simulink model "Controller_damping_cbf_22"  (R2022b)
settings: Solver=ode4  StartTime=0.0  StopTime=Inf  FixedStep=1e-3  RelTol=1e-3
values from neighbouring files (symbols this model uses):
  cbf_damping_params = [cbf_p_ths; cbf_v_ths; cbf_v_0; cbf_gamma; cbf_d_max;                        cbf_w_lin; cbf_w_quad; plane_normal; plane_offset;                        cbf_latch_entry; cbf_zone_hyst; cbf_latch_alpha; cbf_clip_drift;                        cbf_tau_rate; cbf_dt; cbf_gamma_pos_scale]    [init_damping_cbf.m]
  Dn = 20 * ones(7,1)    [init_damping_cbf.m]
  H_0_cy = H_0_pr * H_pr_cy    [init_damping_cbf.m]
  H_home = getTransform(Franka_robot, q_home, 'panda_link8', 'panda_link0')    [init_damping_cbf.m]
  Kn = 0 * ones(7,1)    [init_damping_cbf.m]
  q_home = q_init    [init_damping_cbf.m]
  q_init = [0 0  0  -(2/4)*pi  0  pi/2  -pi/4]'    [init_damping_cbf.m]
undefined symbols (not defined in the file or in its folder): DiscIntNeverNeededParam, Fext_mag, T_final, X, Y, Z
libraries: sm_lib x162, nesl_utility x44, matrix_library x3, Robotics_lib x1
(part 7 of 12)

== matlab function Controller_damping_cbf_22/Dynamic Parameters/Mass Matrix ==
  data: q input; m output
function m = maple_R7plus_massmatrix_04(q)
% Author: TU Wien, ACIN Robotics group
% Optimized and generated from Maple
  m = zeros(7,7);
  t378 = q(6);
  t364 = sin(t378);
  t371 = cos(t378);
  t494 = 0.60149e-1 * t364 - 0.14117e-1 * t371;
  t246 = t494 + 0.384e0;
  t380 = q(4);
  t366 = sin(t380);
  t214 = t246 * t366;
  t381 = q(3);
  t374 = cos(t381);
  t269 = 0.60149e-1 * t371 + 0.14117e-1 * t364;
  t379 = q(5);
  t365 = sin(t379);
  t372 = cos(t379);
  t159 = t269 * t365 + 0.10517e-1 * t372;
  t367 = sin(t381);
  t424 = t159 * t367;
  t373 = cos(t380);
  t681 = 0.10517e-1 * t365;
  t437 = -t269 * t372 + t681;
  t906 = 0.825e-1 + t437;
  t915 = t906 * t373;
  t937 = t424 + (t214 + t915) * t374;
  t377 = q(7);
  t363 = sin(t377);
  t370 = cos(t377);
  t499 = -0.10517e-1 * t370 - 0.4252e-2 * t363;
  t254 = -t499 + 0.88e-1;
  t417 = t254 * t364 - 0.61597e-1 * t371;
  t910 = 0.384e0 + t417;
  t889 = t910 * t366;
  t472 = -0.825e-1 + t889;
  t172 = 0.10517000000000000000000000000000e-1 * t363 - 0.42520000000000000000000000000000e-2 * t370;
  t815 = t172 * t365;
  t682 = 0.61597e-1 * t364;
  t768 = t371 * t372;
  t911 = -t254 * t768 - t372 * t682 + 0.825e-1;
  t70 = -t815 + t911;
  t41 = t373 * t70 + t472;
  t802 = t254 * t371;
  t418 = t682 + t802;
  t895 = t365 * t418;
  t864 = -t172 * t372 + t895;
  t935 = t367 * t864 + t374 * t41;
  t515 = 0.12009367848960000000000000000000e-2 * t363 + 0.63347540234880000000000000000000e-1;
  t530 = 0.29704261916160000000000000000000e-2 * t370;
  t126 = t515 + t530;
  t349 = t363 ^ 2;
  t294 = 0.13297872941088000000000000000000e-4 * t349;
  t356 = t370 ^ 2;
  t328 = 0.2407645905580142000000000000000e-2 * t356;
  t305 = 0.55042935974400000000000000000000e-3 * t363;
  t514 = t305 + 0.57804776249276620000000000000000e-2;
  t459 = -t328 + t294 + t514;
  t562 = 0.79021743663150400000000000000000e-3 * t363;
  t811 = (-0.13614453378240000000000000000000e-2 + t562) * t370;
  t871 = t811 - t459;
  t59 = t871 * t364;
  t928 = -t126 + t59;
  t933 = t371 * t928;
  t916 = t906 * t366;
  t434 = 0.98827089590400000000000000000000e-3 * t363 + 0.52129746651620000000000000000000e-1;
  t138 = 0.24444132201840000000000000000000e-2 * t370 + t434;
  t832 = t138 * t364;
  t358 = t372 ^ 2;
  t316 = 0.24890000000000000000000000000000e-2 * t356;
  t799 = t363 * t370;
  t488 = 0.85600000000000000000000000000000e-3 * t799;
  t453 = t316 + t488;
  t420 = t453 - 0.27050000000000000000000000000000e-2;
  t117 = t453 + 0.28220000000000000000000000000000e-2;
  t357 = t371 ^ 2;
  t99 = t117 * t357;
  t413 = t420 + t99;
  t298 = 0.14820000000000000000000000000000e-2 * t363;
  t532 = 0.23920000000000000000000000000000e-2 * t370;
  t465 = t298 - t532;
  t163 = -t465 + 0.218e-3;
  t796 = t364 * t371;
  t734 = t163 * t796;
  t909 = t734 - t413;
  t932 = t909 * t358;
  t295 = 0.29704261916160000000000000000000e-2 * t363;
  t509 = 0.23898270415101870000000000000000e-1 - t295;
  t535 = 0.12009367848960000000000000000000e-2 * t370;
  t131 = t509 + t535;
  t318 = 0.79021743663150400000000000000000e-3 * t356;
  t238 = -0.68072266891200000000000000000000e-3 * t363 + 0.29134980109706700000000000000000e-3;
  t812 = (0.24209437785212300000000000000000e-2 * t363 + 0.27521467987200000000000000000000e-3) * t370;
  t922 = t238 + t812;
  t908 = -t318 + t922;
  t925 = t908 * t364;
  t698 = t131 + t925;
  t382 = q(2);
  t375 = cos(t382);
  t757 = t375 * t373;
  t368 = sin(t382);
  t772 = t368 * t374;
  t249 = t366 * t772 + t757;
  t804 = t249 * t371;
  t780 = t367 * t368;
  t758 = t375 * t366;
  t761 = t373 * t374;
  t242 = -0.1e1 * t368 * t761 + t758;
  t896 = t242 * t372;
  t140 = t365 * t780 + t896;
  t828 = t140 * t364;
  t919 = -0.1e1 * t828 + t804;
  t351 = t365 ^ 2;
  t792 = t365 * t372;
  t622 = 0.4234e-2 * t792;
  t931 = 0.29474e-1 * t351 + 0.35549e-1 * t358 + t622 + 0.25853e-1;
  t930 = 0.28179e-1;
  t929 = t373 - 0.1e1;
  t927 = t159 * t374;
  t781 = t366 * t374;
  t692 = 0.4252e-2 * t370;
  t500 = 0.10517e-1 * t363 - t692;
  t456 = t500 * t372;
  t399 = t456 - t895;
  t926 = t399 * t367;
  t924 = t908 * t365;
  t923 = t908 * t371;
  t344 = 0.345563e0 * t366;
  t329 = -0.825e-1 + t344;
  t493 = 0.41065e-1 * t365 + 0.11953e-1 * t372;
  t247 = t493 + 0.825e-1;
  t805 = t247 * t373;
  t142 = t329 + t805;
  t173 = -0.41065000000000000000000000000000e-1 * t372 + 0.11953000000000000000000000000000e-1 * t365;
  t73 = t142 * t367 + t173 * t374;
  t748 = t294 + t305;
  t921 = -0.32797153116247448000000000000000e-1 - t748 + t811;
  t383 = q(1);
  t376 = cos(t383);
  t756 = t375 * t376;
  t719 = t367 * t756;
  t369 = sin(t383);
  t770 = t369 * t374;
  t920 = -t719 - t770;
  t725 = t372 * t780;
  t808 = t242 * t365;
  t124 = t808 - 0.1e1 * t725;
  t807 = t246 * t373;
  t918 = t366 * t437 - t807;
  t917 = t59 - t515;
  t304 = 0.63817750210500000000000000000000e-3 * t363;
  t542 = 0.25801376238000000000000000000000e-3 * t370;
  t433 = 0.55993270925625000000000000000000e-2 + t542;
  t127 = -t304 + t433;
  t106 = t127 * t373;
  t540 = 0.54835910640823200000000000000000e-3 * t370;
  t560 = 0.16724826617837780000000000000000e-2 * t363;
  t175 = -t540 - t560;
  t141 = -t175 + 0.9356909731460500000000000000000e-4;
  t824 = t141 * t371;
  t226 = 0.56786982094425000000000000000000e-2 * t364 - 0.12089329343850000000000000000000e-2;
  t183 = t226 * t373;
  t793 = t365 * t371;
  t912 = -0.24076459055801420000000000000000e-2 * t356 - t811;
  t58 = (-0.89033153705875550000000000000000e-2 - t748 - t912) * t357;
  t299 = 0.12763550042100000000000000000000e-2 * t363;
  t541 = 0.51602752476000000000000000000000e-3 * t370;
  t432 = 0.11198654185125000000000000000000e-1 + t541;
  t882 = t299 - t432;
  t891 = t882 * t365;
  t559 = 0.23920000000000000000000000000000e-2 * t363;
  t259 = 0.682e-3 + t559;
  t533 = 0.14820000000000000000000000000000e-2 * t370;
  t265 = t364 * t533;
  t486 = 0.49780000000000000000000000000000e-2 * t799;
  t426 = 0.14600000000000000000000000000000e-2 - t486;
  t565 = 0.17120000000000000000000000000000e-2 * t356;
  t119 = t426 + t565;
  t840 = t119 * t371;
  t914 = t259 * t364 + t265 + t840;
  t700 = 0.825e-1 * t366;
  t704 = 0.825e-1 * t375;
  t913 = t368 * t700 + t704 * t761;
  t68 = t328 + t921;
  t487 = 0.24890000000000000000000000000000e-2 * t799;
  t567 = 0.85600000000000000000000000000000e-3 * t356;
  t116 = t487 - 0.73000000000000000000000000000000e-3 - t567;
  t538 = 0.74100000000000000000000000000000e-3 * t370;
  t483 = t364 * t538;
  t54 = -0.4234e-2 + t914;
  t451 = -0.11960000000000000000000000000000e-2 * t363 - 0.341e-3;
  t686 = t451 * t364 + 0.3449e-2;
  t907 = t116 * t371 + t358 * t54 - t792 * t909 - t483 + t686;
  t400 = -t365 * t500 - t372 * t418;
  t215 = 0.48418875570424600000000000000000e-2 * t363 + 0.55042935974400000000000000000000e-3;
  t561 = 0.13614453378240000000000000000000e-2 * t363;
  t566 = 0.15804348732630080000000000000000e-2 * t356;
  t87 = t215 * t370 - t561 - t566 + 0.5826996021941340000000000000000e-3;
  t78 = t87 * t371;
  t580 = -0.3030488946654060e-2 - t78;
  t534 = 0.12763550042100000000000000000000e-2 * t370;
  t310 = 0.11357396418885000000000000000000e-1 * t364;
  t513 = t310 - 0.24178658687700000000000000000000e-2;
  t313 = 0.56786982094425000000000000000000e-2 * t366;
  t422 = t313 - 0.21751134959804000000000000000000e-1 * t373;
  t306 = 0.54835910640823200000000000000000e-3 * t363;
  t511 = 0.44842466056464210000000000000000e-2 - t306;
  t548 = 0.12089329343850000000000000000000e-2 * t366;
  t904 = 0.46305794820080000000000000000000e-2 * t373 - t511 - t548 + (t422 - 0.26431758938496000000000000000000e-1) * t364;
  t350 = t364 ^ 2;
  t308 = 0.31228377456598930000000000000000e-2 * t350;
  t564 = 0.25022978729410880000000000000000e-2 * t356;
  t427 = t308 + 0.6284682367054690000000000000000e-3 - t564;
  t264 = t370 * t562;
  t293 = 0.81354094419858000000000000000000e-4 * t349;
  t751 = t264 + t293;
  t79 = -t427 + t751;
  t903 = t58 + t79;
  t901 = t54 * t792;
  t572 = 0.2489000000000000000000000000000e-2 * t356;
  t415 = -t488 - t572;
  t120 = -t415 + 0.28220000000000000000000000000000e-2;
  t327 = 0.4978000000000000000000000000000e-2 * t356;
  t263 = 0.17120000000000000000000000000000e-2 * t799;
  t508 = 0.33106000000000000000000000000000e-1 - t263;
  t46 = -t120 * t357 + t327 - t508 + t734;
  t854 = t901 + t932;
  t900 = t46 + t854;
  t169 = -0.825e-1 + t214;
  t884 = t169 + t915;
  t899 = t374 * t884 + t424;
  t537 = 0.10967182128164640000000000000000e-2 * t370;
  t558 = 0.33449653235675560000000000000000e-2 * t363;
  t423 = t537 + t558;
  t405 = t423 + 0.18713819462921000000000000000000e-3;
  t898 = -t364 * t405 - t580;
  t464 = 0.33449653235675560000000000000000e-2 * t370 - 0.10967182128164640000000000000000e-2 * t363;
  t128 = 0.11022068765350630000000000000000e-1 + t464;
  t108 = t128 * t357;
  t555 = 0.88000000000000000000000000000000e-1 * t364;
  t224 = 0.38400000000000000000000000000000e0 + t555;
  t897 = t224 * t367;
  t490 = -0.104419e0 * t373 + 0.5317e-1 * t366;
  t893 = t368 * t490;
  t645 = 0.345563e0 * t373;
  t806 = t247 * t366;
  t576 = -t645 + t806;
  t892 = t368 * t576;
  t721 = t374 * t756;
  t779 = t367 * t369;
  t503 = t373 * (t721 - 0.1e1 * t779);
  t890 = (t576 - 0.316e0) * t375;
  t822 = t910 * t373;
  t222 = -t304 + 0.55993270925625000000000000000000e-2;
  t888 = (t222 + t542) * t373;
  t492 = -0.41065e-1 * t372 + 0.11953e-1 * t365;
  t887 = t492 * t367;
  t623 = 0.7735484874e-2 * t370;
  t154 = (0.76800000000000000000000000000000e0 * t364 + 0.17600000000000000000000000000000e0) * t623;
  t231 = 0.24018735697920000000000000000000e-2 * t363 + 0.12669508046976000000000000000000e0;
  t885 = t231 * t364 + t154;
  t326 = 0.54835910640823200000000000000000e-3 * t374;
  t543 = 0.24444132201840000000000000000000e-2 * t367;
  t881 = t326 + t543;
  t595 = 0.2964e-2 * t363 - 0.4784e-2 * t370 - 0.436e-3;
  t880 = -0.1e1 * t328 - 0.26431758938496000000000000000000e-1 * t371 - t921;
  t879 = t363 * t681 - t365 * t692 - t911;
  t877 = t514 + t912;
  t648 = 0.249498e0 * t368;
  t679 = 0.39252e-1 * t367;
  t876 = -t375 * t679 + t648;
  t627 = 0.3127439544e-2 * t363;
  t875 = t623 + t627;
  t874 = 0.88e-1 * t371 + t682;
  t740 = t128 * t796;
  t873 = t740 - t58;
  t870 = t58 - 0.1e1 * t740;
  t258 = -0.74100000000000000000000000000000e-3 * t363 + 0.4146e-2;
  t536 = 0.11960000000000000000000000000000e-2 * t370;
  t737 = t120 * t796;
  t818 = t163 * t357;
  t439 = -t536 + t737 + t818;
  t869 = -0.1e1 * t258 + t439;
  t568 = t263 + 0.5644000000000000000000000000000e-2;
  t121 = t327 + t568;
  t736 = t121 * t796;
  t463 = -0.47840000000000000000000000000000e-2 * t370 + 0.29640000000000000000000000000000e-2 * t363;
  t162 = t463 - 0.436e-3;
  t819 = t162 * t357;
  t867 = t736 - 0.1e1 * t819;
  t322 = 0.13614453378240000000000000000000e-2 * t370;
  t866 = -0.1e1 * t305 - 0.1e1 * t322;
  t649 = 0.104419e0 * t366;
  t491 = 0.5317e-1 * t373 + t649;
  t248 = t491 - 0.825e-1;
  t442 = t248 * t367;
  t669 = 0.27454e-1 * t374;
  t865 = (t442 + t669) * t376;
  t863 = 0.735522e0 * t369;
  t647 = 0.735522e0 * t371;
  t657 = 0.27518e-1 * t369;
  t660 = 0.39252e-1 * t376;
  t862 = t376 * t648 + (-t375 * t660 - t657) * t367;
  t795 = t364 * t372;
  t861 = -t116 * t795 - 0.8641e-2;
  t860 = 0.1225946e1 * t73;
  t296 = 0.24444132201840000000000000000000e-2 * t363;
  t431 = 0.98827089590400000000000000000000e-3 * t370 + 0.21447119530300000000000000000000e-1;
  t139 = -t296 + t431;
  t225 = -0.21751134959804000000000000000000e-1 * t364 + 0.46305794820080000000000000000000e-2;
  t859 = t139 * t365 + (-0.1e1 * t138 * t371 + t225) * t372;
  t858 = 0.25801376238000000000000000000000e-3 * t366 - 0.98827089590400000000000000000000e-3;
  t563 = 0.25801376238000000000000000000000e-3 * t363;
  t234 = 0.13609823097337500000000000000000e-1 + t563;
  t539 = 0.63817750210500000000000000000000e-3 * t370;
  t132 = t234 + t539;
  t111 = t132 * t364;
  t857 = 0.29682175996164750000000000000000e0 + t111;
  t856 = 0.47796540830203740000000000000000e-1 - 0.59408523832320000000000000000000e-2 * t363;
  t855 = -t364 * t534 + 0.11357396418885000000000000000000e-1 * t371;
  t516 = t249 * t364;
  t827 = t140 * t371;
  t80 = t516 + t827;
  t853 = t370 * t80;
  t443 = -0.81354094419858e-4 * t356 - 0.89033153705875550000000000000000e-2;
  t747 = t305 + t322;
  t90 = t294 - t443 + t747;
  t852 = t373 * t90;
  t851 = ((t294 + t877) * t357 + t740 - 0.22516878283212450000000000000000e-2) * t351;
  t47 = (-0.1e1 * t811 + t459) * t364 + t126;
  t850 = t47 * t371;
  t846 = t80 * t363;
  t664 = 0.10517e-1 * t376;
  t606 = t375 * t664;
  t670 = 0.10517e-1 * t374;
  t201 = -t367 * t606 - t369 * t670;
  t677 = 0.10517e-1 * t369;
  t204 = -t367 * t677 + t374 * t606;
  t613 = t368 * t664;
  t843 = t201 * t793 + (-t204 * t366 + t373 * t613) * t364;
  t688 = 0.4252e-2 * t376;
  t760 = t374 * t375;
  t211 = t688 * t760 - 0.4252e-2 * t779;
  t620 = t368 * t688;
  t690 = 0.4252e-2 * t371;
  t842 = t920 * t365 * t690 + (-t211 * t366 + t373 * t620) * t364;
  t841 = (t316 + t264 + 0.31228377456598930000000000000000e-2) * t350;
  t839 = t124 * t363;
  t838 = t124 * t370;
  t837 = t127 * t366;
  t223 = -0.51602752476000000000000000000000e-3 * t363 - 0.27219646194675000000000000000000e-1;
  t130 = -t223 + t534;
  t836 = t130 * t371;
  t112 = t132 * t366;
  t835 = t132 * t373;
  t547 = 0.82500000000000000000000000000000e-1 * t366;
  t227 = -0.38400000000000000000000000000000e0 + t547;
  t135 = t227 - 0.31600000000000000000000000000000e0 * t373;
  t834 = t135 * t371;
  t137 = t231 + 0.59408523832320000000000000000000e-2 * t370;
  t833 = t137 * t364;
  t831 = t138 * t373;
  t829 = t139 * t373;
  t826 = t141 * t364;
  t825 = t141 * t365;
  t823 = t142 * t374;
  t146 = t423 + 0.187138194629210e-3;
  t821 = t146 * t364;
  t817 = (t259 + t533) * t371;
  t165 = -t451 + t538;
  t816 = t165 * t371;
  t813 = t173 * t367;
  t177 = (0.18713819462921000000000000000000e-3 + t558) * t364;
  t810 = t222 * t366;
  t239 = 0.9356909731460500000000000000000e-4 + t560;
  t191 = t239 * t364;
  t809 = t239 * t374;
  t297 = 0.15804348732630080000000000000000e-2 * t363;
  t800 = t297 * t370;
  t798 = t364 * t365;
  t797 = t364 * t367;
  t794 = t365 * t367;
  t791 = t365 * t373;
  t790 = t365 * t374;
  t789 = t365 * t375;
  t788 = t366 * t364;
  t787 = t366 * t365;
  t786 = t366 * t367;
  t785 = t366 * t368;
  t784 = t366 * t371;
  t783 = t366 * t372;
  t782 = t366 * t373;
  t777 = t367 * t373;
  t776 = t367 * t374;
  t775 = t367 * t375;
  t774 = t367 * t376;
  t773 = t368 * t373;
  t769 = t369 * t375;
  t767 = t371 * t373;
  t766 = t371 * t374;
  t765 = t371 * t375;
  t764 = t372 * t373;
  t763 = t372 * t375;
  t762 = t373 * t364;
  t759 = t374 * t376;
  t713 = 0.88e-1 * t376;
  t635 = t374 * t713;
  t715 = 0.88e-1 * t367;
  t637 = t369 * t715;
  t213 = -t375 * t635 + t637;
  t636 = t368 * t713;
  t755 = t213 * t366 + t373 * t636;
  t311 = 0.35079000000000000000000000000000e-3 * t365;
  t235 = -0.92549600000000000000000000000000e-3 - t311;
  t754 = t235 * t373 + t311;
  t519 = 0.10517000000000000000000000000000e-1 * t376;
  t753 = t519 * t775 + 0.10517000000000000000000000000000e-1 * t770;
  t315 = 0.49780000000000000000000000000000e-2 * t356;
  t752 = t263 + t315;
  t750 = t264 + t328;
  t702 = 0.825e-1 * t376;
  t342 = t374 * t702;
  t290 = t375 * t342;
  t347 = 0.316e0 * t368;
  t341 = t376 * t347;
  t749 = t290 + t341;
  t705 = 0.825e-1 * t374;
  t337 = t368 * t705;
  t746 = -t337 + 0.316e0 * t375;
  t745 = -0.1e1 * t373 + 0.1e1;
  t266 = t364 * t537;
  t744 = t78 - t177 - t266;
  t743 = t373 * t841;
  t125 = -0.21800000000000000000000000000000e-3 + t465;
  t742 = t125 * t796;
  t741 = t374 * t108;
  t97 = t128 * t762;
  t275 = 0.8074e-2 * t372 + 0.458e-3 * t365;
  t739 = t275 * t782;
  t738 = t358 * t758;
  t735 = t162 * t796;
  t732 = t165 * t793;
  t731 = t365 * t763;
  t730 = t366 * t841;
  t729 = t128 * t788;
  t728 = t371 * t758;
  t727 = t366 * t757;
  t726 = t367 * t769;
  t724 = t371 * t764;
  t723 = t372 * t761;
  t722 = t369 * t760;
  t720 = t376 * t785;
  t709 = 0.825e-1 * t369;
  t633 = t367 * t709;
  t718 = t373 * t633 + t749;
  t717 = -t347 + t913;
  t716 = -t375 * t700 + t746;
  t712 = 0.428e-3 * t363;
  t711 = 0.109e-3 * t364;
  t710 = 0.384e0 * t366;
  t708 = 0.384e0 * t369;
  t707 = 0.428e-3 * t370;
  t706 = 0.109e-3 * t371;
  t703 = 0.384e0 * t375;
  t701 = 0.384e0 * t376;
  t321 = 0.16724826617837780000000000000000e-2 * t370;
  t129 = t321 + t511;
  t309 = 0.26431758938496000000000000000000e-1 * t364;
  t93 = -t309 - t129;
  t699 = -t93 - t108;
  t697 = 0.1482e-2 * t363;
  t695 = 0.4252e-2 * t368;
  t694 = 0.1482e-2 * t370;
  t693 = 0.2392e-2 * t370;
  t689 = 0.3495e-2 * t376;
  t279 = t366 * t613;
  t685 = t204 * t373 + t279;
  t574 = -0.1e1 * t802 - t682;
  t69 = t864 * t374;
  t683 = 0.735522e0 * (t367 * t472 + t70 * t777 - t69) * t376 + (t935 * t375 - 0.1e1 * t347 + (-t822 + (0.825e-1 - 0.1e1 * t815 + t574 * t372) * t366) * t368) * t863;
  t680 = 0.27454e-1 * t367;
  t678 = 0.61597e-1 * t367;
  t676 = 0.14117e-1 * t369;
  t675 = 0.27454e-1 * t369;
  t674 = 0.39252e-1 * t369;
  t673 = 0.60149e-1 * t369;
  t668 = 0.27518e-1 * t374;
  t667 = 0.39252e-1 * t374;
  t666 = 0.61597e-1 * t374;
  t665 = 0.10517e-1 * t375;
  t663 = 0.14117e-1 * t376;
  t662 = 0.27454e-1 * t376;
  t661 = 0.27518e-1 * t376;
  t659 = 0.60149e-1 * t376;
  t658 = 0.61597e-1 * t376;
  t270 = 0.2872e-1 * t375 + 0.3141e-2 * t368;
  t654 = 0.646926e0 * t270;
  t72 = -t823 + t813;
  t653 = 0.1225946e1 * (t72 * t375 + t347 + (-0.1e1 * t806 + t645) * t368) * t376 + t369 * t860;
  t88 = -t887 + t823;
  t652 = 0.1225946e1 * (t375 * t88 - t347 + t892) * t369 + t376 * t860;
  t594 = t807 - t916;
  t651 = 0.1666555e1 * (t594 + 0.316e0) * t375 + 0.1666555e1 * t899 * t368;
  t650 = 0.735522e0 * t363;
  t81 = t367 * t661 + t369 * t876 + t374 * t660 + t657 * t760;
  t643 = 0.3228604e1 * t81;
  t579 = t248 * t374 - t680;
  t642 = -0.3587895e1 * t579 * t368 + 0.3587895e1 * (t490 - 0.316e0) * t375;
  t338 = t369 * t347;
  t630 = t367 * t702;
  t639 = t369 * t913 + t373 * t630 - t338;
  t631 = t374 * t703;
  t287 = t366 * t631;
  t638 = t287 + t717;
  t634 = t367 * t708;
  t632 = t369 * t704;
  t340 = t368 * t701;
  t629 = 0.3127439544e-2 * t224;
  t628 = 0.7735484874e-2 * t224;
  t626 = 0.3127439544e-2 * t365;
  t625 = 0.7735484874e-2 * t365;
  t624 = 0.3127439544e-2 * t370;
  t621 = t367 * t695;
  t619 = 0.15592e-1 * t782;
  t618 = t369 * t678;
  t616 = 0.10517e-1 * t780;
  t615 = t368 * t676;
  t614 = t368 * t673;
  t612 = t368 * t663;
  t611 = t368 * t659;
  t610 = t368 * t658;
  t609 = t369 * t665;
  t608 = t375 * t676;
  t607 = t375 * t673;
  t605 = t375 * t663;
  t604 = t375 * t659;
  t603 = t375 * t658;
  t601 = t375 * t661;
  t600 = 0.735522e0 * t781;
  t599 = t340 * t373 + t366 * t634 + t718;
  t343 = 0.13297872941088e-4 * t356;
  t331 = 0.2392e-2 * t363 + 0.682e-3;
  t596 = t331 + t694;
  t591 = t373 * t629;
  t228 = -0.31600000000000000000000000000000e0 + t547;
  t590 = t228 * t623;
  t589 = -t699 + t933;
  t588 = t287 * t369 + t701 * t786 + t639;
  t587 = t290 - t633;
  t586 = t721 - t779;
  t585 = t726 - t759;
  t267 = t364 * t540;
  t584 = t267 + t191 + 0.2390110552949070e-2;
  t583 = -0.1e1 * t788 + t724;
  t582 = t726 - 0.1e1 * t759;
  t578 = -0.1e1 * t770 - 0.1e1 * t719;
  t577 = -0.1e1 * t722 - 0.1e1 * t774;
  t575 = t367 * t632 - t342;
  t573 = -0.1e1 * t79 + t873;
  t571 = 0.4841887557042460000000000000000e-2 * t356;
  t570 = 0.5483591064082320000000000000000e-3 * t371;
  t569 = 0.5483591064082320000000000000000e-3 * t374;
  t556 = 0.49096519673609460000000000000000e-2 * t364;
  t554 = 0.86765250000000000000000000000000e-3 * t365;
  t553 = 0.42520000000000000000000000000000e-2 * t365;
  t552 = 0.49096519673609460000000000000000e-2 * t365;
  t550 = 0.54835910640823200000000000000000e-3 * t366;
  t549 = 0.63817750210500000000000000000000e-3 * t366;
  t546 = 0.25801376238000000000000000000000e-3 * t367;
  t545 = 0.63817750210500000000000000000000e-3 * t367;
  t544 = 0.16724826617837780000000000000000e-2 * t367;
  t529 = 0.16724826617837780000000000000000e-2 * t371;
  t528 = 0.54835910640823200000000000000000e-3 * t372;
  t527 = 0.25801376238000000000000000000000e-3 * t373;
  t526 = 0.54835910640823200000000000000000e-3 * t373;
  t525 = 0.63817750210500000000000000000000e-3 * t373;
  t524 = 0.16724826617837780000000000000000e-2 * t373;
  t523 = 0.49096519673609460000000000000000e-2 * t373;
  t522 = 0.10517000000000000000000000000000e-1 * t373;
  t517 = 0.21751134959804000000000000000000e-1 * t371;
  t512 = 0.12089329343850000000000000000000e-2 * t929;
  t510 = -0.23044843893347959000000000000000e-1 - t293;
  t507 = -0.65941286852573577000000000000000e0 - t305;
  t505 = t266 + t580;
  t504 = t373 * t582;
  t502 = 0.2872e-1 * t368 - 0.3141e-2 * t375;
  t498 = t365 * t577;
  t497 = t366 * t578;
  t496 = t578 * t373;
  t495 = (t59 - 0.1e1 * t126) * t372 + t825;
  t489 = -t668 + t679;
  t485 = t364 * t546;
  t484 = t364 * t545;
  t482 = 0.49096519673609460000000000000000e-2 * t784;
  t481 = t364 * t526;
  t480 = t364 * t524;
  t479 = t372 * t523;
  t147 = t343 - t510;
  t236 = -t559 - 0.68200000000000000000000000000000e-3;
  t474 = t236 * t364 - t265 + 0.42340000000000000000000000000000e-2;
  t471 = t373 * t575 + t585 * t710 - t575;
  t104 = (-t368 * t702 - t376 * t631 + t634) * t366;
  t470 = (t340 - t587) * t373 + t104 + t341 + t587;
  t469 = 0.56786982094425000000000000000000e-2 * t745;
  t237 = -0.37417600000000000000000000000000e-3 + t554;
  t468 = t237 * t373 - t554;
  t460 = t364 * t486;
  t452 = -0.1e1 * t316 - t488;
  t450 = -0.8292e-2 - t532;
  t449 = t309 + t321 + 0.44842466056464210000000000000000e-2 - t108 - 0.1e1 * t306;
  t448 = t318 - 0.1e1 * t812;
  t446 = -0.1712e-2 * t356 + 0.4978e-2 * t799 - 0.1460e-2;
  t445 = 0.4978e-2 * t356 + 0.1712e-2 * t799 + 0.5644e-2;
  t444 = t365 * t589 + 0.1644487577369270e-2;
  t50 = t925 + (t239 + t540) * t371;
  t436 = -t374 * t491 + t680;
  t430 = 0.26431758938496000000000000000000e-1 * t373 + 0.21751134959804000000000000000000e-1;
  t429 = t366 * t493 - t645;
  t156 = t368 * t489 + 0.249498e0 * t375;
  t428 = t264 + 0.2502297872941088000000000000000e-2 * t356 - 0.60029938106866070000000000000000e-2;
  t176 = 0.16724826617837780000000000000000e-2 * t374 + 0.98827089590400000000000000000000e-3 * t367;
  t414 = t373 * t493 + t329;
  t412 = t535 + 0.23898270415101870000000000000000e-1 + (-0.1e1 * t318 + t922) * t364;
  t408 = 0.42520000000000000000000000000000e-2 * t920;
  t407 = t129 * t373 + (-t313 + t430) * t364 + t548 - 0.46305794820080000000000000000000e-2;
  t406 = -t373 * t628 + t549 - 0.24444132201840000000000000000000e-2;
  t403 = (0.104419e0 * t368 - 0.5317e-1 * t760) * t373 + (-0.104419e0 * t760 - 0.5317e-1 * t368) * t366;
  t401 = (-t835 + t132) * t372 + t97;
  t398 = t375 * t579 + t893;
  t397 = t366 * t494 + t373 * t437 - 0.825e-1;
  t396 = t887 + (-t344 - t805) * t374;
  t395 = t367 * t414 + t374 * t492;
  t394 = -t400 - 0.825e-1;
  t393 = t367 * t397 - t927;
  t392 = t429 * t368 + (t374 * t414 - t887) * t375;
  t391 = t366 * t400 - t822;
  t390 = t366 * t417 + t373 * t400 - 0.825e-1;
  t389 = (-0.1e1 * t816 + 0.229e-3) * t372 + t869 * t365 + t861;
  t388 = t918 * t368 + (t374 * t397 + t424) * t375;
  t387 = t367 * t390 + t374 * t399;
  t386 = t926 + (t373 * t394 - t889) * t374;
  t385 = 0.27752814537092170000000000000000e0 + ((0.66899306471351120000000000000000e-2 * t370 - 0.21934364256329280000000000000000e-2 * t363 + 0.22044137530701260000000000000000e-1) * t357 + (((t297 - 0.27228906756480000000000000000000e-2) * t370 - 0.26595745882176000000000000000000e-4 * t349 + 0.4815291811160284000000000000000e-2 * t356 - 0.11008587194880000000000000000000e-2 * t363 - 0.11560955249855324000000000000000e-1) * t364 - t137) * t371 - 0.52863517876992000000000000000000e-1 * t364 - 0.8968493211292842000000000000000e-2 - t464) * t372;
  t384 = t391 * t368 + (t374 * t390 - t926) * t375;
  t360 = t374 ^ 2;
  t359 = t373 ^ 2;
  t353 = t367 ^ 2;
  t352 = t366 ^ 2;
  t335 = t369 * t669;
  t323 = 0.21751134959804000000000000000000e-1 * t372;
  t314 = 0.54835910640823200000000000000000e-3 * t367;
  t291 = t366 * t636;
  t281 = t366 * t620;
  t280 = t374 * t601;
  t278 = t366 * t610;
  t274 = -0.8074e-2 * t365 + 0.458e-3 * t372;
  t260 = 0.14600000000000000000000000000000e-2 * t364 + 0.458e-3;
  t253 = t375 * t662 - t709;
  t252 = t375 * t702 + t675;
  t251 = t375 * t675 + t702;
  t250 = t632 - t662;
  t244 = t519 * t785;
  t243 = t565 * t798;
  t232 = -0.31600000000000000000000000000000e0 * t366 + 0.82500000000000000000000000000000e-1;
  t229 = 0.82500000000000000000000000000000e-1 * t929;
  t212 = t375 * t637 - t635;
  t209 = t695 * t761 - 0.4252e-2 * t758;
  t208 = -t367 * t609 + t374 * t664;
  t207 = t366 * t665 - t670 * t773;
  t206 = -t367 * t603 - t369 * t666;
  t205 = t374 * t603 - t618;
  t203 = -t367 * t676 + t374 * t605;
  t202 = -t367 * t673 + t374 * t604;
  t200 = t367 * t605 + t374 * t676;
  t199 = t367 * t604 + t374 * t673;
  t198 = -t367 * t664 - t374 * t609;
  t197 = t367 * t663 + t374 * t608;
  t196 = t367 * t659 + t374 * t607;
  t195 = -t367 * t608 + t374 * t663;
  t194 = -t367 * t607 + t374 * t659;
  t193 = t374 * t658 - t375 * t618;
  t192 = t239 * t367;
  t185 = t234 * t366;
  t182 = t226 * t366;
  t174 = -t321 + t306;
  t171 = -0.12150e-1 * t792 - 0.4234e-2 * t351 + 0.4234e-2 * t358;
  t161 = t376 * t502 - 0.3495e-2 * t369;
  t153 = t227 * t623;
  t148 = -0.93569097314605e-4 + t175;
  t136 = -t228 + 0.38400000000000000000000000000000e0 * t373;
  t134 = -0.26431758938496000000000000000000e-1 * t366 - 0.56786982094425000000000000000000e-2 * t929;
  t114 = t141 * t372;
  t94 = -t135 + t555;
  t74 = t908 * t762;
  t71 = (-0.68072266891200000000000000000000e-3 * t370 - 0.27521467987200000000000000000000e-3 * t363 - 0.49096519673609460000000000000000e-2) * t371 + t174 * t364;
  t61 = (t205 * t366 + 0.88e-1 * t365 * t578 - t373 * t610) * t371;
  t51 = -t295 + t412;
  t48 = 0.3030488946654060e-2 + t744;
  t34 = ((-0.68072266891200000000000000000000e-3 * t364 + t529 - 0.29704261916160000000000000000000e-2) * t370 + (-0.54835910640823200000000000000000e-3 * t371 - 0.27521467987200000000000000000000e-3 * t364 - 0.12009367848960000000000000000000e-2) * t363 - t556) * t365 + (-0.25801376238000000000000000000000e-3 * t364 + (-0.12009367848960000000000000000000e-2 * t371 - 0.54835910640823200000000000000000e-3) * t372) * t370 + (0.63817750210500000000000000000000e-3 * t364 + (0.29704261916160000000000000000000e-2 * t371 - 0.16724826617837780000000000000000e-2) * t372) * t363;
  t31 = 0.15592e-1 + (t298 + t450 + t867) * t372 - 0.1e1 * t243 + (t817 + t460 - 0.1e1 * t260) * t365;
  t28 = t880 * t372 + (-t132 - t924) * t371 + (t126 * t372 + t825 - 0.56786982094425000000000000000000e-2) * t364;
  t24 = (t449 - t933) * t365 + (t698 + t824) * t372;
  t23 = ((t174 * t371 + t224 * t875 + t556) * t372 + (0.28244044800000000000000000000000e0 * t172 * t371 + t175) * t365) * t366 + (t468 * t650 - 0.1e1 * t523) * t371 + t363 * t481 - 0.735522e0 * t499 * t229 * t372 + (-0.1e1 * t480 + t754 * t647) * t370;
  t22 = ((t126 * t364 + t880) * t365 + (-0.1e1 * t826 + t923) * t372) * t366 + ((t229 * t623 + t234 * t373 - t234) * t364 + t371 * t469) * t365 + t74 + t370 * t371 * t526 + t239 * t767;
  t15 = (((-t371 * t524 - t406) * t372 + (-0.4252e-2 * t136 * t365 + 0.92549600000000000000000000000000e-3 * t366) * t647 - t365 * t526) * t370 + ((t373 * t570 + t591 - t858) * t372 + (t136 * t681 + 0.37417600000000000000000000000000e-3 * t366) * t647 - t365 * t524) * t363 + t482) * t367 + (((-0.3127439544e-2 * t834 + 0.54835910640823200000000000000000e-3) * t372 - t365 * t529 + t94 * t625) * t370 + ((0.7735484874e-2 * t834 + 0.16724826617837780000000000000000e-2) * t372 + t365 * t570 + t94 * t626) * t363) * t374 + ((t321 * t366 - t363 * t550 + t479) * t367 + ((0.3127439544e-2 * t232 - t527) * t370 + (-0.7735484874e-2 * t232 + t525) * t363 + t552) * t374) * t364;
  t14 = t147 * t373 + t357 * t852 + t401 * t371 + t743 + (t364 * t469 + t366 * t589 + t512) * t372 + ((t50 + t131) * t366 + t888 - 0.1e1 * t542 - 0.1e1 * t222) * t365;
  t13 = (-t127 * t372 + t358 * t48 + t584 - t923) * t366 + ((t824 - 0.1e1 * t295 + t412) * t372 - 0.1644487577369270e-2) * t373 + ((t573 * t372 - 0.1e1 * t132 * t371 - 0.1e1 * t226) * t366 + (-0.1e1 * t108 + t850 - 0.1e1 * t93) * t373) * t365;
  t12 = (((-0.1e1 * t138 * t372 - 0.56786982094425000000000000000000e-2) * t373 + (t227 * t627 + t153 - 0.63347540234880000000000000000000e-1) * t372 - 0.1e1 * t825 + 0.56786982094425000000000000000000e-2) * t364 + ((-0.1e1 * t132 + t323) * t373 + (-0.1e1 * t313 + 0.26431758938496000000000000000000e-1) * t372 + t924 + 0.13609823097337500000000000000000e-1 + t875 * t232) * t371 + t68 * t372) * t374 + (((t126 * t365 - t114) * t373 + (-t228 * t627 - t590 + 0.52129746651620000000000000000000e-1) * t365) * t364 + ((t372 * t908 - 0.26431758938496000000000000000000e-1 * t365) * t373 + (t313 - 0.21751134959804000000000000000000e-1) * t365) * t371 - t68 * t791) * t367 + (((0.13609823097337500000000000000000e-1 * t372 - 0.21751134959804000000000000000000e-1) * t364 - 0.52129746651620000000000000000000e-1 * t371) * t374 + ((-t238 - 0.13609823097337500000000000000000e-1 * t365 + t448) * t364 - t824) * t367) * t366;
  t9 = ((((t176 * t373 - 0.1e1 * t366 * t546 + 0.12009367848960000000000000000000e-2 * t367) * t371 + t314 + t406 * t374) * t372 + (t235 * t600 + (-0.1e1 * t544 + (0.12009367848960000000000000000000e-2 * t373 + 0.98827089590400000000000000000000e-3) * t374) * t365) * t371 + (t881 * t365 - 0.1e1 * t485) * t373 + (-0.1e1 * t176 * t364 - 0.1e1 * t365 * t545) * t366 + t625 * t897 + t485) * t370 + (((-0.1e1 * t373 * t569 + (-0.24444132201840000000000000000000e-2 * t373 + t549 - 0.29704261916160000000000000000000e-2) * t367) * t371 + t544 + (-0.1e1 * t591 + t858) * t374) * t372 + (t237 * t600 + (t314 + (-0.29704261916160000000000000000000e-2 * t373 - 0.24444132201840000000000000000000e-2) * t374) * t365) * t371 + (t176 * t365 + t484) * t373 + (t881 * t364 - 0.1e1 * t365 * t546) * t366 + t626 * t897 - 0.1e1 * t484) * t363 - 0.1e1 * t364 * t374 * t479 - 0.1e1 * t374 * t482 + t552 * t797) * t368 + (0.49096519673609460000000000000000e-2 * t364 * t783 - 0.49096519673609460000000000000000e-2 * t767 + ((t366 * t628 + t525 - 0.63817750210500000000000000000000e-3) * t372 + (-0.16327680000000000000000000000000e-2 * t787 + t754) * t647 - 0.1e1 * t365 * t550 - 0.1e1 * t529 * t783 - 0.1e1 * t480) * t370 + ((t366 * t629 + t527 - 0.25801376238000000000000000000000e-3) * t372 + (0.40385280000000000000000000000000e-2 * t787 + t468) * t647 - 0.16724826617837780000000000000000e-2 * t787 + t528 * t784 + t481) * t363) * t375;
  t8 = (t764 * t108 + ((t185 - 0.1e1 * t434 + t590) * t372 - 0.1e1 * t729 + t495 * t373) * t371 - 0.1e1 * t407 * t372 + (t131 * t373 - 0.1e1 * t228 * t624 - 0.1e1 * t296 + t74 - 0.1e1 * t810 + 0.21447119530300000000000000000000e-1) * t365 - 0.1e1 * t730 + ((-0.1e1 * t294 + t443 + t866) * t357 - 0.1e1 * t343 + t510) * t366) * t367 + t365 * t741 + (-t114 + (t153 + t185 - t831 + t917) * t365) * t766 + ((t227 * t624 - t509 + t810 - t829 - t925) * t372 + (-t321 + t904) * t365) * t374;
  t7 = (((-0.1e1 * t314 * t370 - 0.1e1 * t192 + (-0.1e1 * t126 * t373 + t112 - t138) * t374) * t365 + (-0.56786982094425000000000000000000e-2 * t367 + ((-0.1e1 * t543 + t569) * t370 - t434 * t367 + t809) * t372) * t373 + ((t132 * t372 - 0.21751134959804000000000000000000e-1) * t367 + t908 * t374) * t366 + (-t372 * t515 + 0.56786982094425000000000000000000e-2) * t367) * t364 + (t367 * t923 + ((-0.1e1 * t313 + t430) * t371 + t68 * t373) * t374) * t365 + ((t326 * t370 + t809) * t366 + (0.7902174366315040000000000000000e-3 * t356 - 0.1e1 * t812 - 0.1e1 * t238) * t723 + ((t323 - 0.13609823097337500000000000000000e-1) * t373 + (-0.56786982094425000000000000000000e-2 * t372 - 0.1e1 * t138) * t366 + 0.26431758938496000000000000000000e-1 * t372 + 0.13609823097337500000000000000000e-1 + (t539 + t563) * t745) * t367) * t371) * t368 + t375 * ((t126 * t366 + t835 - 0.1e1 * t132) * t365 + t908 * t373 - 0.1e1 * t141 * t783) * t364 + (t134 * t371 - t366 * t68) * t789 + (t141 * t373 + t783 * t908) * t765 + (-0.1e1 * t530 * t364 + t68) * t725;
  t6 = (-t371 * t835 - t183) * t794 + ((t293 + t428) * t358 + (t898 * t365 + (-t835 + t130) * t371 - t183 + t513) * t372 + t851 + (t106 + t882) * t365 + (-0.1e1 * t313 + 0.52863517876992000000000000000000e-1) * t371 - 0.1e1 * t833 - 0.65941286852573577000000000000000e0 + t866) * t374 + (((-0.1e1 * t824 - t698) * t372 + t444) * t367 + (t857 + t859) * t374) * t366 + ((t898 * t358 + (t573 * t365 - 0.1e1 * t127) * t372 - t923 + t826 + 0.2390110552949070e-2) * t367 + (t517 - 0.1e1 * t832 - 0.50330438027992300000000000000000e0) * t374) * t373;
  t5 = ((t90 * t781 + (-0.1e1 * t723 + t794) * t128) * t357 + (-0.1e1 * t192 * t372 + ((-0.1e1 * t112 + t138) * t372 + t729 + (-t928 * t372 - 0.1e1 * t825) * t373) * t374 + (-0.1e1 * t370 * t528 + (t112 - 0.1e1 * t831 - 0.1e1 * t530 + t917) * t365) * t367) * t371 + (t407 * t374 + ((-0.1e1 * t238 + t448) * t364 - 0.1e1 * t829 + t837 - 0.1e1 * t535 - t509) * t367) * t372 + ((t837 + (-t925 - 0.1e1 * t131) * t373 - 0.1e1 * t139) * t374 + (-0.1e1 * t321 + t904) * t367) * t365 + t374 * t730 + t147 * t781) * t368 + (t366 * t495 + t401) * t765 + (-0.1e1 * t129 * t366 + t134 * t364 + t512) * t763 + (t698 * t366 + t106 - 0.1e1 * t127) * t789 + t147 * t757 + ((t128 * t783 + t852) * t357 + t743) * t375;
  t4 = (-0.36044563611157510600000000000000e0 + ((t146 * t365 - 0.11357396418885000000000000000000e-1) * t371 + (t87 * t364 + 0.24018735697920000000000000000000e-2 * t370 + t856) * t365 + t130 * t364 + t385) * t359 + (0.56786982094425000000000000000000e-2 * t371 - 0.1e1 * t111 + 0.12908973617152500000000000000000e-1 + t859) * t373 + ((-0.1e1 * t112 - t928) * t371 - 0.1e1 * t182 + t449) * t372 + (t148 * t365 + 0.56786982094425000000000000000000e-2) * t371 - t698 * t365 - 0.1e1 * t111 + (((t564 - 0.1e1 * t308 - 0.28801560650267140000000000000000e-2 + t751 + t870) * t358 + ((t365 * t87 + t130) * t371 + (-0.1e1 * t821 + 0.3030488946654060e-2) * t365 + t513) * t372 + (-0.1e1 * t294 + 0.2489553776598930000000000000000e-3 + t750) * t357 + (-0.1e1 * t128 * t364 - 0.52863517876992000000000000000000e-1) * t371 - 0.22516878283212450000000000000000e-2 * t351 + t891 + (0.60294330025875550000000000000000e-2 + t747) * t350 + t833 - 0.1e1 * t571 - 0.1e1 * t800 + 0.54361295502067749900000000000000e0) * t373 - 0.1e1 * t517 + t127 * t365 + t832 + 0.58416762559717300000000000000000e0) * t366) * t367 + ((t148 * t371 - t698) * t372 + t444) * t761 + ((t132 * t365 + t908) * t366 - 0.1e1 * t138 * t365) * t766 + t225 * t790 + ((t580 + t821) * t358 + t148 * t364 + t226 * t365 - 0.2390110552949070e-2) * t781 + (((-0.1e1 * t304 + (t79 + t870) * t365 + t433) * t366 - 0.1e1 * t139) * t372 - 0.13297019103287584000000000000000e-1) * t374;
  t3 = (((-0.1096718212816464e-2 * t370 - 0.3344965323567556e-2 * t363 - 0.187138194629210e-3) * t797 * t365 + t781 * t824 + (-0.1e1 * t97 * t793 + t106 + t51 * t366) * t374) * t372 + (t835 * t766 + (-0.1e1 * t741 + t47 * t766 - 0.1e1 * t93 * t374) * t366) * t365 - 0.16444875773692700000000000000000e-2 * t781 - 0.1e1 * t231 * t797 + ((t505 + t177) * t358 + t923 - 0.1e1 * t191 - 0.1e1 * t267 - 0.23901105529490700000000000000000e-2 + (t372 * t903 + t226) * t365) * t761) * t368 + t48 * t738 + ((t51 + t824) * t373 + ((-0.1e1 * t264 - 0.1e1 * t293 + t427 + t873) * t365 - 0.1e1 * t127) * t366) * t763 + (-0.1e1 * t112 * t371 - 0.1e1 * t182 + (t699 + t850) * t373) * t789 - 0.1e1 * t908 * t728 - 0.1644487577369270e-2 * t757 + t584 * t758 + ((0.2502297872941088e-2 * t356 + 0.790217436631504e-3 * t799 - 0.6002993810686607e-2 + t293) * t358 + (((-0.1580434873263008e-2 * t356 + (0.4841887557042460e-2 * t363 + 0.55042935974400000000000000000000e-3) * t370 - 0.1e1 * t561 + 0.582699602194134e-3) * t371 + 0.3030488946654060e-2) * t365 + (-0.1e1 * t835 - t138 * t366 + t534 - 0.1e1 * t223) * t371 - 0.1e1 * t183 + t225 * t366 + t513) * t372 + t851 + (t888 - 0.1e1 * t541 + t299 - 0.11198654185125000000000000000000e-1 + (-0.1e1 * t296 + t431) * t366) * t365 + (-0.1e1 * t422 + 0.52863517876992000000000000000000e-1) * t371 + (-t832 - 0.50330438027992300000000000000000e0) * t373 + t857 * t366 - 0.1e1 * t154 + t507) * t780;
  t2 = ((t657 + 0.39252000000000000000000000000000e-1 * t756) * t374 + (0.27518000000000000000000000000000e-1 * t756 - 0.1e1 * t674) * t367) * t643 + 0.3228604e1 * ((-0.39252000000000000000000000000000e-1 * t367 + t668) * t376 + (-0.27518000000000000000000000000000e-1 * t367 - 0.1e1 * t667) * t769) * ((-0.27518e-1 * t367 - 0.1e1 * t667) * t369 + t280 + t876 * t376) + (t73 * t756 + (-0.1e1 * t813 + t823) * t369) * t652 + (t376 * t72 + t73 * t769) * t653 + ((t367 * t41 - 0.1e1 * t69) * t756 + t935 * t369) * t683 + 0.735522e0 * (((t371 * t685 + t408) * t372 + (-0.1e1 * t720 + (-0.1e1 * t721 + t779) * t373) * t553 + t843) * t370 + (((t211 * t373 + t281) * t371 + t753) * t372 + (t244 + 0.10517000000000000000000000000000e-1 * t503) * t365 + t842) * t363 + ((t205 * t373 + t278) * t372 + t206 * t365 + t755) * t364 + (-0.1e1 * t213 * t373 + t291) * t768 + t61 + t470) * ((t198 * t793 + t208 * t583 + 0.42520000000000000000000000000000e-2 * t372 * t577 + t504 * t553) * t370 + (-0.4252e-2 * t583 * t585 + t498 * t690 + 0.10517000000000000000000000000000e-1 * (t722 + t774) * t372 + (-0.1e1 * t726 + t759) * t365 * t522) * t363 + (t193 * t764 + t212 * t366 + 0.61597e-1 * t498) * t364 - 0.1e1 * t212 * t724 + (t193 * t366 + 0.88e-1 * t498) * t371 + t471) + ((t367 * t389 + t781 * t900) * t373 - 0.12805000000000000000000000000000e-1 * t367 + (-0.1e1 * t567 + t487) * t364 * t790 + t907 * t786 + (((-0.1e1 * t736 + t819 - 0.1e1 * t298 - 0.1e1 * t450) * t372 + t243 - 0.15592e-1 + (-0.1e1 * t817 - 0.1e1 * t460 + t260) * t365) * t359 + t869 * t372 + t732 + 0.19192000000000000000000000000000e-1 + (-0.73000000000000000000000000000000e-3 * t364 - 0.229e-3) * t365) * t374) * t368 + t31 * t727 + (-0.1e1 * t840 + t474) * t352 * t731 + (t46 * t359 + (t413 + t742) * t352 * t358 + 0.84106000000000000000000000000000e-1 - 0.1e1 * t572 - 0.1e1 * t488) * t375 + 0.3587895e1 * (-0.1e1 * t253 * t374 + t252 * t367 + 0.104419e0 * t497 + 0.5317e-1 * t496) * (t250 * t374 + t338 + (-0.1e1 * t491 * t376 + t251) * t367 + t403 * t369) + 0.3587895e1 * (t252 * t374 + t341 + (t369 * t491 + t253) * t367 + t403 * t376) * (t251 * t374 - 0.1e1 * t250 * t367 + t582 * t649 + 0.5317e-1 * t504) + 0.1666555e1 * ((t199 * t764 + t200 * t366 + t202 * t365) * t371 + (t200 * t764 - 0.1e1 * t199 * t366 + t203 * t365) * t364 + t201 * t791 + t204 * t372 + 0.384e0 * t497 + 0.825e-1 * t496 + t375 * t630 + t369 * t705) * ((t194 * t365 + (t196 * t373 + t366 * t614) * t372 + t197 * t366 - 0.1e1 * t373 * t615) * t371 + (t195 * t365 + (t197 * t373 + t366 * t615) * t372 - 0.1e1 * t196 * t366 + t373 * t614) * t364 + (t198 * t373 - 0.1e1 * t677 * t785) * t365 + t208 * t372 + t338 + t708 * t773 + t577 * t710 + t745 * t630 + (-0.1e1 * t785 + t745 * t760) * t709) + 0.1666555e1 * ((-0.1e1 * t199 * t365 + (t202 * t373 + t366 * t611) * t372 + t203 * t366 - 0.1e1 * t373 * t612) * t371 + (-0.1e1 * t200 * t365 + (t203 * t373 + t366 * t612) * t372 - 0.1e1 * t202 * t366 + t373 * t611) * t364 - 0.1e1 * t685 * t365 + t201 * t372 + t470) * ((t194 * t764 + t195 * t366 - 0.1e1 * t196 * t365) * t371 + (-0.1e1 * t194 * t366 + t195 * t764 - 0.1e1 * t197 * t365) * t364 - 0.1e1 * t208 * t791 + t198 * t372 + t471);
  t1 = ((((t279 + 0.10517e-1 * t503) * t371 + t408) * t372 + (-0.1e1 * t586 * t373 - 0.1e1 * t720) * t553 + t843) * t370 + ((t281 * t371 + t503 * t690 + t753) * t372 + (t522 * t586 + t244) * t365 + t842) * t363 + (t278 * t364 + t291 * t371 + t503 * t874) * t372 + t61 + t206 * t798 + t755 * t364 + t104 + (t373 - 0.1e1) * t633 + (t340 - 0.1e1 * t290) * t373 + t749) * (((t207 * t371 + t621) * t372 + t209 * t365 + t616 * t793 + 0.10517e-1 * t516) * t370 + ((-0.1e1 * t616 - 0.1e1 * t209 * t371) * t372 + t207 * t365 + t621 * t793 + 0.4252e-2 * t516) * t363 + (t365 * t368 * t715 - 0.1e1 * t666 * t785 - 0.61597e-1 * t757) * t371 + t368 * t678 * t798 + 0.88e-1 * t516 + (0.384e0 * t772 - 0.1e1 * t704) * t366 + (t337 + t703) * t373 + t746 + t874 * t896) * t863 + (0.95220000000000000000000000000000e-2 + (-0.6898e-2 + ((0.99560000000000000000000000000000e-2 * t799 - 0.34240000000000000000000000000000e-2 * t356 - 0.29200000000000000000000000000000e-2) * t371 + 0.8468e-2 + (-0.47840000000000000000000000000000e-2 * t363 - 0.29640000000000000000000000000000e-2 * t370 - 0.1364e-2) * t364) * t358 + (0.5410000000000000000000000000000e-2 + (-0.1e1 * t315 - 0.1e1 * t568) * t357 - 0.1e1 * t735 - 0.1e1 * t752) * t792 + t914) * t373 + (t119 * t364 - 0.1e1 * t817 + 0.458e-3) * t783 + (-0.17282e-1 + (t298 - 0.8292e-2) * t365) * t366 + (-0.1e1 * t532 + t867) * t787) * t368 * t360 + ((t900 * t359 + t31 * t782 + t121 * t357 + t735 + 0.31784000000000000000000000000000e-1 + t415 + t854) * t780 + t389 * t757 + t54 * t738 - t366 * t909 * t731 + t116 * t728 - 0.1e1 * t483 * t758 + (t686 * t366 - 0.12805000000000000000000000000000e-1) * t375) * t374 + (-0.15015000000000000000000000000000e-1 + t907 * t373 + ((-0.229e-3 + t816) * t372 + (-0.1e1 * t818 - 0.1e1 * t737 + t536 + t258) * t365 - 0.1e1 * t861) * t366) * t368 - 0.704e-3 * t375 + ((-t932 - 0.1e1 * t46 - 0.1e1 * t901) * t727 + (-0.1e1 * t439 + t258) * t763) * t367 + (t31 * t359 - 0.1e1 * t732 - 0.19192000000000000000000000000000e-1 + (-0.1e1 * t116 * t364 + 0.229e-3) * t365) * t775 + (t161 * t654 + 0.3228604e1 * t156 * ((t601 - 0.1e1 * t674) * t374 + t862) - 0.1e1 * (t248 * t779 + t335) * t642 - 0.1e1 * ((-0.1e1 * t823 + t887) * t368 + t890) * t653 + (-0.1e1 * t159 * t770 + 0.1e1 * t906 * t369 * t777 + t169 * t779) * t651) * t369 + (-0.1e1 * t689 * t654 - 0.1e1 * t156 * t643 - 0.1e1 * t865 * t642 + (t88 * t368 - 0.1e1 * t890) * t652 - 0.1e1 * ((t373 * t879 - t472) * t772 + (-0.1e1 * t879 * t366 - t822 - 0.316e0) * t375 + (t365 * t574 + t456) * t780) * t683 + (-0.1e1 * t927 + t884 * t367) * t651 * t376 + (-0.1e1 * t502 * t654 + ((t899 + (-t915 - 0.1e1 * t214 + 0.825e-1) * t374 - 0.1e1 * t424) * t375 + (0.1e1 * t916 - 0.1e1 * t807 + t594) * t368) * t651) * t369) * t376;
  m(7,7) = 0.49096519673609460000000000000000e-2;
  m(2,4) = t6;
  m(6,4) = t28;
  m(4,3) = t13;
  m(7,4) = t34;
  m(7,6) = t175;
  m(6,7) = t175;
  m(3,3) = 0.68731045565809253900000000000000e0 + ((-t740 + t903) * t358 + (0.30304889466540600000000000000000e-2 + t744) * t792 - 0.52863517876992000000000000000000e-1 * t371 + t305 + 0.10771188545559324000000000000000e-1 + t885) * t352 + ((-0.1e1 * t566 * t798 + (0.70158000000000000000000000000000e-3 * t650 + 0.27219646194675000000000000000000e-1) * t364 + t385 + (t405 * t371 + (t215 * t364 + 0.24018735697920000000000000000000e-2) * t370 + (-0.18509920000000000000000000000000e-2 * t650 + 0.5826996021941340000000000000000e-3) * t364 + t856) * t365 - t855) * t373 + t223 * t364 - 0.28391278634449500000000000000000e0 + t855) * t366 + (-0.53661951164938448500000000000000e0 + (-0.1e1 * t836 - 0.1e1 * t310 + 0.24178658687700000000000000000000e-2) * t372 - t871 * t357 + t740 + t571 + t800 - t891) * t359 + ((t513 + t836) * t372 - 0.80863245317250000000000000000000e-1 + t891) * t373 + t294 - t750;
  m(2,1) = t1;
  m(3,4) = t13;
  m(2,3) = t4;
  m(6,2) = t12;
  m(5,5) = t357 * t90 + t147 + t740 + t841;
  m(6,3) = t22;
  m(7,1) = t9;
  m(7,5) = t71;
  m(4,4) = ((-0.13297872941088e-4 * t349 - t877) * t357 - t740 + 0.2251687828321245e-2) * t351 + (-0.1e1 * t299 + ((0.187138194629210e-3 + t558) * t364 + t505) * t372 + t432) * t365 + (-t130 * t372 - 0.52863517876992000000000000000000e-1) * t371 + (-0.81354094419858e-4 * t349 - t428) * t358 - t513 * t372 - t507 + t885;
  m(4,2) = t6;
  m(4,1) = t3;
  m(5,7) = t71;
  m(5,6) = t50;
  m(1,6) = t7;
  m(5,2) = t8;
  m(5,3) = t14;
  m(7,2) = t15;
  m(4,7) = t34;
  m(3,5) = t14;
  m(2,5) = t8;
  m(1,7) = t9;
  m(1,4) = t3;
  m(3,6) = t22;
  m(3,1) = t2;
  m(3,2) = t4;
  m(4,5) = t24;
  m(2,2) = 0.646926e0 * t502 ^ 2 + 0.3228604e1 * (t375 * t489 - t648) ^ 2 + 0.3587895e1 * (-t347 + t398) ^ 2 + 0.1225946e1 * (t392 + t717) ^ 2 + 0.1666555e1 * (t388 + t638) ^ 2 + 0.735522e0 * (t384 + t638) ^ 2 + 0.103407e0 + ((t117 * t358 * t359 + t366 * (-0.43600000000000000000000000000000e-3 + t463) * t764) * t357 + ((t125 * t358 * t364 - 0.1e1 * t119 * t792) * t359 + ((-0.56440000000000000000000000000000e-2 - 0.1e1 * t315 - 0.1e1 * t263) * t795 + (t236 - 0.1e1 * t533) * t365) * t782) * t371 + (t358 * t420 + t474 * t792 - 0.1e1 * t315 + t508) * t359 + ((t532 + 0.82920000000000000000000000000000e-2 - 0.1e1 * t298) * t372 + t243 - 0.15592000000000000000000000000000e-1 + (0.45800000000000000000000000000000e-3 + t426 * t364) * t365) * t782 + t453) * t353 + (-0.9522e-2 + t365 * ((0.5644e-2 + t752) * t764 + t595 * t366) * t357 + (((0.2920e-2 + 0.3424e-2 * t356 - 0.9956e-2 * t799) * t358 + t364 * t595 * t792 + t446) * t373 + (t596 * t372 - 0.1e1 * t445 * t798) * t366) * t371 + (0.6898e-2 - 0.8468e-2 * t358 + (-0.5410e-2 + t752) * t792 + ((0.4784e-2 * t363 + 0.2964e-2 * t370 + 0.1364e-2) * t358 - 0.1e1 * t694 - 0.1e1 * t331) * t364) * t373 + (t446 * t364 - 0.458e-3) * t783 + t693 * t787 + (0.17282e-1 + (0.8292e-2 - 0.1e1 * t697) * t365) * t366) * t776 + (0.31784e-1 + ((-0.2822e-2 - 0.2489e-2 * t356 - 0.856e-3 * t799) * t359 + (-0.2822e-2 + t452) * t358 + t445) * t357 + (0.2705e-2 + t452) * t358 + (-0.1e1 * t446 * t371 - 0.4234e-2) * t792 + ((t595 + (t358 + t359) * (t693 + 0.218e-3 - 0.1e1 * t697)) * t371 + t596 * t792) * t364) * t360 + (-0.1e1 * t99 - 0.1e1 * t742) * t352 + (t369 ^ 2 + t376 ^ 2) * (0.3228604e1 * t156 ^ 2 + 0.735522e0 * (t368 * t386 + t375 * t391 - t716) ^ 2 + 0.1666555e1 * (t368 * t937 - t375 * t918 + t716) ^ 2 + 0.1225946e1 * (-t368 * t396 - t375 * t429 + t716) ^ 2 + 0.3587895e1 * (t368 * t436 + t375 * t490 - t746) ^ 2 + 0.646926e0 * t270 ^ 2);
  m(4,6) = t28;
  m(1,1) = (-0.4354e-2 * t828 + 0.4354e-2 * t804 + t140 * t706 + t249 * t711 + 0.341e-3 * t124) * t919 + (-0.5433e-2 * t725 + 0.5433e-2 * t808 - 0.1158e-2 * t827 - 0.1158e-2 * t516 + 0.341e-3 * t919) * t124 + (0.12516e-1 * t839 + 0.12516e-1 * t853 - 0.1e1 * t124 * t707 + t80 * t712 + 0.1196e-2 * t919) * (t839 + t853) + (0.10027e-1 * t838 - 0.10027e-1 * t846 - 0.1e1 * t124 * t712 - 0.1e1 * t80 * t707 + 0.741e-3 * t919) * (-0.1e1 * t846 + t838) + (0.1964e-2 * t827 + 0.1964e-2 * t516 - 0.1e1 * t140 * t711 + t249 * t706 + 0.1158e-2 * t725 - 0.1158e-2 * t808) * t80 + 0.17079e-1 + (0.4815e-2 * t828 - 0.4815e-2 * t804 - 0.1196e-2 * t839 - 0.1196e-2 * t853 - 0.741e-3 * t838 + 0.741e-3 * t846) * (t828 - 0.1e1 * t804) + 0.4970684e1 * (-0.3875e-2 * t369 - 0.2081e-2 * t376) ^ 2 + 0.4970684e1 * (0.3875e-2 * t376 - 0.2081e-2 * t369) ^ 2 + 0.3587895e1 * (t369 * t398 - t338 + t865) ^ 2 + 0.3587895e1 * (t335 + t369 * t442 + (t375 * t436 - t893) * t376 + t749) ^ 2 + 0.3228604e1 * t81 ^ 2 + 0.3228604e1 * (-t369 * t667 + t280 + t862) ^ 2 + 0.1666555e1 * (t393 * t369 + ((t373 * t494 - t916) * t368 - t937 * t375) * t376 + t599) ^ 2 + 0.1666555e1 * (t369 * t388 + t376 * t393 + t588) ^ 2 + 0.1225946e1 * (t369 * t392 + t376 * t395 + t639) ^ 2 + 0.1225946e1 * (t395 * t369 + (t375 * t396 - t892) * t376 + t718) ^ 2 + 0.735522e0 * (t369 * t384 + t376 * t387 + t588) ^ 2 + 0.735522e0 * (t387 * t369 + ((t366 * t394 + t373 * t417) * t368 + t386 * t375) * t376 + t599) ^ 2 + 0.646926e0 * (-t369 * t502 - t689) ^ 2 + 0.646926e0 * t161 ^ 2 + (-0.1e1 * t739 + 0.30978000000000000000000000000000e-1 + t619 + t930 * t359 + t931 * t352) * t375 ^ 2 + ((-0.1e1 * (-0.2664e-2 * t366 + 0.17282e-1 * t373) * t367 + t274 * t777 - 0.1e1 * t171 * t786 - 0.7850e-2 - 0.25610000000000000000000000000000e-1 * t367 + (0.22792000000000000000000000000000e-1 + (-0.15592e-1 + t275) * (t359 - 0.1e1 * t352) + (0.4652e-2 - 0.58948e-1 * t351 - 0.71098e-1 * t358 - 0.8468e-2 * t792) * t782) * t374) * t375 + (0.36155000000000000000000000000000e-1 + (0.28323e-1 + 0.35549e-1 * t351 + 0.29474e-1 * t358 - 0.1e1 * t622) * t353 + (0.95220000000000000000000000000000e-2 + (-0.2664e-2 + t171) * t373 + (-0.17282e-1 + t274) * t366) * t776 + (-0.1e1 * t619 + 0.1087000000000000000000000000000e-2 + t739 + t931 * t359 + t930 * t352) * t360) * t368) * t368;
  m(5,1) = t5;
  m(6,6) = -0.2420943778521230000000000000000e-2 * t356 + (-t562 + 0.1361445337824e-2) * t370 + 0.550429359744e-3 * t363 + 0.32810450989188536000000000000000e-1;
  m(5,4) = t24;
  m(2,6) = t12;
  m(2,7) = t15;
  m(6,5) = t50;
  m(1,5) = t5;
  m(1,3) = t2;
  m(1,2) = t1;
  m(6,1) = t7;
  m(7,3) = t23;
  m(3,7) = t23;
end
